simulink model "visionx_telemedicine"  (R2026a)
settings: Solver=VariableStepAuto  StopTime=21600
settings Model: Creator=iPC  LastModifiedBy=iPC

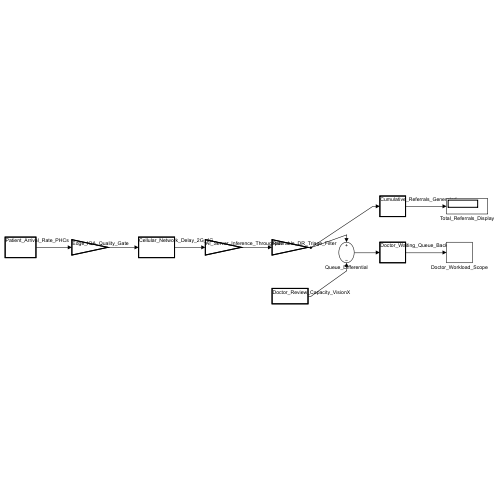
[thumbnail: Simulink's stored preview of the top-level diagram]
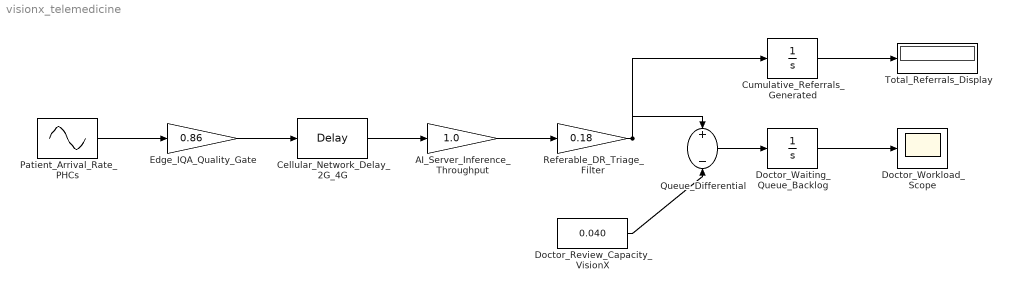
== system visionx_telemedicine ==
  AI_Server_Inference_Throughput : Gain  Gain=1.0
  Cellular_Network_Delay_2G_4G : TransportDelay  DelayTime=1.2
  Cumulative_Referrals_Generated : Integrator
  Doctor_Review_Capacity_VisionX : Constant  Value=0.040
  Doctor_Waiting_Queue_Backlog : Integrator  LimitOutput=on  LowerSaturationLimit=0
  Doctor_Workload_Scope : Scope
  Edge_IQA_Quality_Gate : Gain  Gain=0.86
  Patient_Arrival_Rate_PHCs : Sin  Amplitude=0.012  Bias=0.037  Frequency=0.00029  SampleTime=1
  Queue_Differential : Sum  Inputs=+-
  Referable_DR_Triage_Filter : Gain  Gain=0.18
  Total_Referrals_Display : Display
  wires:
  Patient_Arrival_Rate_PHCs/1 -> Edge_IQA_Quality_Gate/1
  Edge_IQA_Quality_Gate/1 -> Cellular_Network_Delay_2G_4G/1
  Cellular_Network_Delay_2G_4G/1 -> AI_Server_Inference_Throughput/1
  AI_Server_Inference_Throughput/1 -> Referable_DR_Triage_Filter/1
  Referable_DR_Triage_Filter/1 -> Cumulative_Referrals_Generated/1, Queue_Differential/1
  Cumulative_Referrals_Generated/1 -> Total_Referrals_Display/1
  Doctor_Review_Capacity_VisionX/1 -> Queue_Differential/2
  Queue_Differential/1 -> Doctor_Waiting_Queue_Backlog/1
  Doctor_Waiting_Queue_Backlog/1 -> Doctor_Workload_Scope/1
